simulink model "rsw_quad_x"  (Simulink 8.0)
Description:
  | generated by rsw-audit

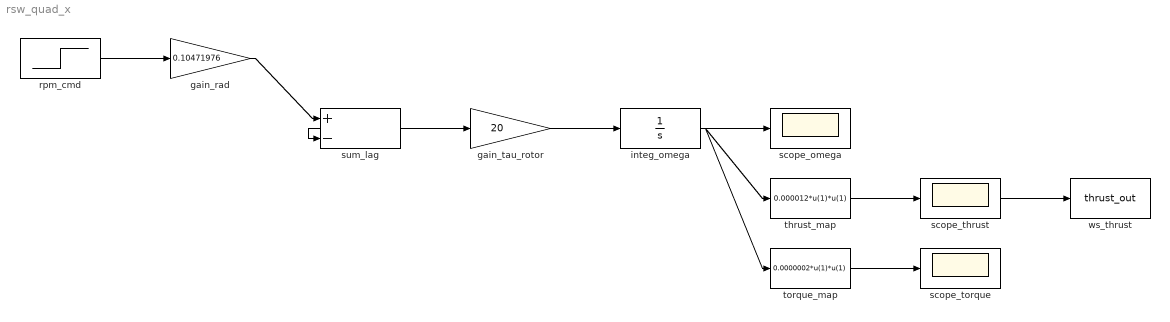
== system rsw_quad_x ==
  rpm_cmd : Step  Time=0  Before=0  After=9000
  gain_rad : Gain  Gain=0.10471976
  sum_lag : Sum  Inputs=+-
  gain_tau_rotor : Gain  Gain=20
  integ_omega : Integrator  InitialCondition=0
  thrust_map : Fcn  Expr=0.000012*u(1)*u(1)
  scope_thrust : Scope
  ws_thrust : ToWorkspace  VariableName=thrust_out  SaveFormat=Array
  scope_omega : Scope
  torque_map : Fcn  Expr=0.0000002*u(1)*u(1)
  scope_torque : Scope
  wires:
  thrust_map/1 -> ws_thrust/1
  integ_omega/1 -> torque_map/1
  torque_map/1 -> scope_torque/1
  rpm_cmd/1 -> gain_rad/1
  gain_rad/1 -> sum_lag/1
  integ_omega/1 -> sum_lag/2
  sum_lag/1 -> gain_tau_rotor/1
  gain_tau_rotor/1 -> integ_omega/1
  integ_omega/1 -> thrust_map/1
  thrust_map/1 -> scope_thrust/1
  integ_omega/1 -> scope_omega/1
